simulink model "screeningWorkflow_review"  (R2026b)
settings: Solver=VariableStepAuto  StopTime=10
settings Model: Creator=azizn  LastModifiedBy=azizn

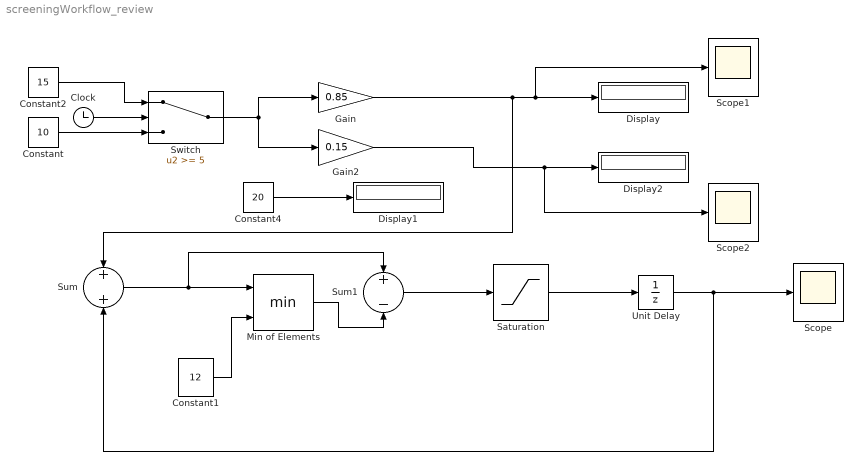
== system screeningWorkflow_review ==
  Clock : Clock
  Constant : Constant  Value=10
  Constant1 : Constant  Value=12
  Constant2 : Constant  Value=15
  Constant4 : Constant  Value=20
  Display : Display
  Display1 : Display
  Display2 : Display
  Gain : Gain  Gain=0.85
  Gain2 : Gain  Gain=0.15
  Min of Elements : MinMax  Inputs=2
  Saturation : Saturate  UpperLimit=inf  LowerLimit=0
  Scope : Scope
      settings: MaximizeAxes=On  ActiveDisplayYMinimum=-26.780923486024587  ActiveDisplayYMaximum=10.28465054615474
  Scope1 : Scope
      settings: MaximizeAxes=On  ActiveDisplayYMinimum=-376.45397224221705  ActiveDisplayYMaximum=441.94471554227556
  Scope2 : Scope
      settings: MaximizeAxes=On  ActiveDisplayYMinimum=-604.97384104084836  ActiveDisplayYMaximum=938.2389426584424  DataLoggingVariableName=ScopeData2
  Sum : Sum
  Sum1 : Sum  Inputs=+-
  Switch : Switch  Threshold=5  SaturateOnIntegerOverflow=off  InputSameDT=off
  Unit Delay : UnitDelay
  wires:
  Constant1/1 -> Min of Elements/2
  Sum1/1 -> Saturation/1
  Saturation/1 -> Unit Delay/1
  Unit Delay/1 -> Sum/2, Scope/1
  Sum/1 -> Sum1/1, Min of Elements/1
  Min of Elements/1 -> Sum1/2
  Constant2/1 -> Switch/1
  Switch/1 -> Gain/1, Gain2/1
  Gain2/1 -> Scope2/1, Display2/1
  Constant4/1 -> Display1/1
  Clock/1 -> Switch/2
  Constant/1 -> Switch/3
  Gain/1 -> Sum/1, Scope1/1, Display/1
